simulink model "Three_blocks_discrete"  (R2017b)
settings: Solver=VariableStepAuto  StartTime=0.0  StopTime=100  RelTol=1e-3
libraries: simulink x3
settings Model: Creator=giuli  LastModifiedBy=giuli

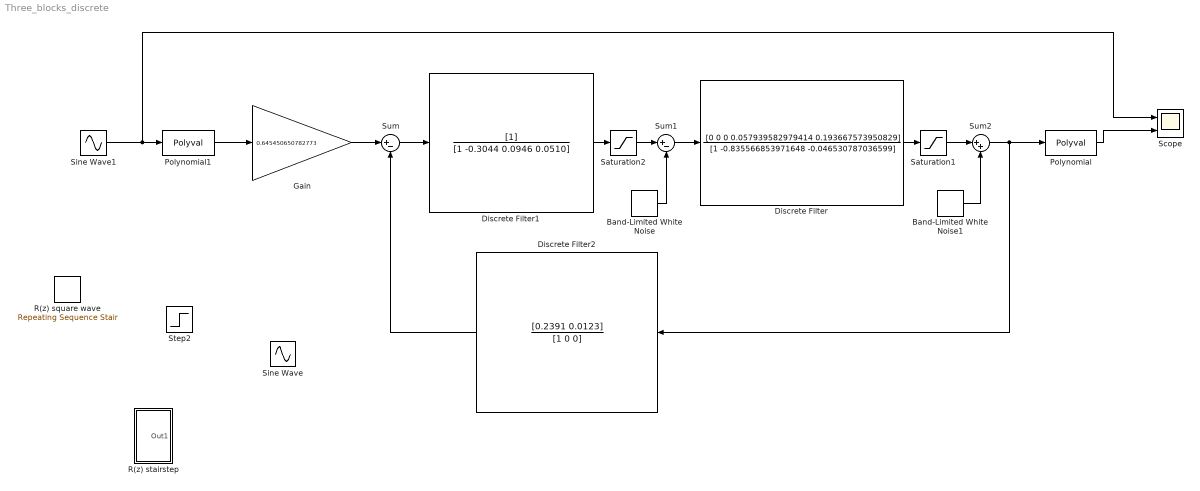
== system Three_blocks_discrete ==
  Band-Limited White Noise : simulink/Sources/Band-Limited White Noise  Cov=[0.01]  Ts=0.08  seed=[23341]
  Band-Limited White Noise1 : simulink/Sources/Band-Limited White Noise  Cov=[0.01]  Ts=0.08  seed=[23341]
  Discrete Filter : DiscreteFilter  Numerator=[0 0 0 0.057939582979414 0.193667573950829]  Denominator=[1 -0.835566853971648 -0.046530787036599]  SampleTime=0.08
  Discrete Filter1 : DiscreteFilter  Denominator=[1 -0.3044 0.0946 0.0510]  SampleTime=0.08
  Discrete Filter2 : DiscreteFilter  Numerator=[0.2391 0.0123]  Denominator=[1 0 0]  SampleTime=0.08
  Gain : Gain  Gain=0.645450650782773
  Polynomial : Polyval  Coefs=[2.865 26.323]
  Polynomial1 : Polyval  Coefs=[1/2.865 -26.323/2.865]
  R(z) square wave : simulink/Sources/Repeating Sequence Stair  OutValues=[15 45 40 30 25 30 40]  tsamp=20  OutMin=[]  OutMax=[]  OutDataTypeStr=double  OutputDataTypeScalingMode=double  OutDataType=fixdt(0,8)  ConRadixGroup=Best Precision: Vector-wise  OutScaling=2^-12
  R(z) stairstep : Subsystem
  Saturation1 : Saturate  UpperLimit=10  LowerLimit=-10
  Saturation2 : Saturate  UpperLimit=5  LowerLimit=0
  Scope : Scope  NumInputPorts=2
  Sine Wave : Sin  Amplitude=10  Bias=35  Frequency=0.1  SampleTime=0
  Sine Wave1 : Sin  Amplitude=10  Bias=35  Frequency=0.1  SampleTime=0
  Step2 : Step  Before=30  After=45  SampleTime=0.08
  Sum : Sum  Inputs=|+-
  Sum1 : Sum  Inputs=|+-
  Sum2 : Sum  Inputs=|++
  wires:
  Sum/1 -> Discrete Filter1/1
  Sine Wave1/1 -> Polynomial1/1, Scope/1
  Gain/1 -> Sum/1
  Polynomial/1 -> Scope/2
  Discrete Filter2/1 -> Sum/2
  Discrete Filter/1 -> Saturation1/1
  Polynomial1/1 -> Gain/1
  Sum1/1 -> Discrete Filter/1
  Band-Limited White Noise/1 -> Sum1/2
  Band-Limited White Noise1/1 -> Sum2/2
  Saturation1/1 -> Sum2/1
  Sum2/1 -> Discrete Filter2/1, Polynomial/1
  Discrete Filter1/1 -> Saturation2/1
  Saturation2/1 -> Sum1/1

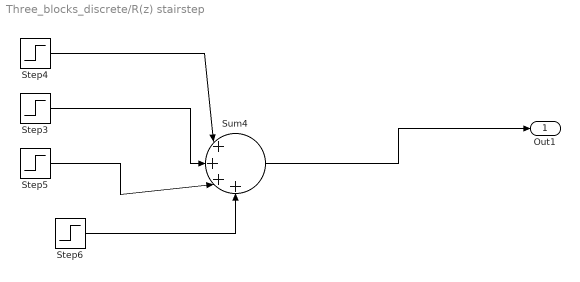
== system Three_blocks_discrete/R(z) stairstep ==
  Step3 : Step  Time=15  Before=30  After=35  SampleTime=0
  Step4 : Step  Time=25  After=5  SampleTime=0
  Step5 : Step  Time=35  After=5  SampleTime=0
  Step6 : Step  Time=45  After=5  SampleTime=0
  Sum4 : Sum  Inputs=|++++
  Out1 : Outport
  wires:
  Step5/1 -> Sum4/3
  Step4/1 -> Sum4/1
  Step6/1 -> Sum4/4
  Step3/1 -> Sum4/2
  Sum4/1 -> Out1/1
